simulink model "I2C_MultipleSequence_FinitStateMachine"  (Simulink 6.4)
settings: Solver=FixedStepDiscrete  StartTime=0.0  StopTime=10.0  FixedStep=0.001  RelTol=1e-3
libraries: dsPICdrivers x6, simulink x3
settings Model: Creator=Lubin  LastModifiedBy=Lubin  ProdHWDeviceType=16-bit Generic
settings OptimizationCC: OptimizeModelRefInitCode=on  LifeSpan=1
settings DebuggingCC: MultiTaskDSMMsg=error  MultiTaskCondExecSysMsg=error
settings HardwareCC: ProdBitPerInt=16  ProdWordSize=16  ProdHWDeviceType=16-bit Generic
settings RTWCC: SystemTargetFile=dspic.tlc  TemplateMakefile=dspic_pic30_gcc.tmf  PostCodeGenCommand=dsPIC_Compile()  Description=Embedded Target for Microchip dsPIC (real-time)  ProcessScript=dspic_make_rtw_hook
settings CodeAppCC: IgnoreCustomStorageClasses=off
settings STFCustomTargetCC: TargetFcnLib=ansi_tfl_tmw.mat  GenFloatMathFcnCalls=ANSI_C  ModelReferenceCompliant=off  IncludeMdlTerminateFcn=off  CombineOutputUpdateFcns=on  SuppressErrorStatus=on  IncludeERTFirstTime=on  ERTFirstTimeCompliant=on  ERTCustomFileBanners=on  SupportContinuousTime=off  SupportNonInlinedSFcns=off  SystemTargetFile=dspic.tlc
settings ERTTargetCC: TargetFcnLib=ansi_tfl_tmw.mat  GenFloatMathFcnCalls=ANSI_C  ModelReferenceCompliant=off  IncludeMdlTerminateFcn=off  SuppressErrorStatus=on  IncludeERTFirstTime=on  InlinedParameterPlacement=NonHierarchical  ERTSrcFileBannerTemplate=dsPIC_code_template.cgt  ERTHdrFileBannerTemplate=dsPIC_code_template.cgt  ERTDataSrcFileTemplate=dsPIC_code_template.cgt  ERTDataHdrFileTemplate=dsPIC_code_template.cgt  ERTCustomFileTemplate=dsPIC_main.tlc  InitialValueSource=Model
settings CustomProperty: DataType=string  Value=C:\PROGRA~1\MATLAB\R2007b\bin\win32\gmake

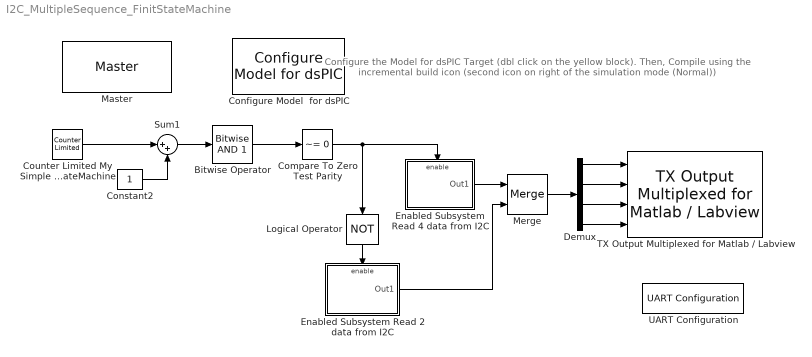
== system I2C_MultipleSequence_FinitStateMachine ==
  note: Configure the Model for dsPIC Target (dbl click on the yellow block).
      | Then, Compile using the incremental build icon
      | (second icon on right of the simulation mode (Normal))
  Bitwise Operator : simulink/Logic and Bit Operations/Bitwise Operator  logicop=AND  UseBitMask=on  BitMask=1  BitMaskRealWorld=Stored Integer
  Compare To Zero Test Parity : simulink/Logic and Bit Operations/Compare To Zero  SystemSampleTime=-1  relop=~=  LogicOutDataTypeMode=uint8  ZeroCross=off
  Configure Model  for dsPIC : dsPICdrivers/Simulink Configuration/Configure Model  for dsPIC
  Constant2 : Constant  Value=1  OutDataTypeMode=uint16  OutDataType=sfix(16)  ConRadixGroup=Use specified scaling  OutScaling=2^0  SampleTime=inf  FramePeriod=inf
  Counter Limited My Simple StateMachine : simulink/Sources/Counter Limited  SystemSampleTime=-1  uplimit=5  tsamp=.001
  Demux : Demux
  Enabled Subsystem Read 2 data from I2C : Subsystem  TreatAsAtomicUnit=on
  Enabled Subsystem Read 4 data from I2C : Subsystem  TreatAsAtomicUnit=on
  Logical Operator : Logic  Orientation=down  Operator=NOT  AllPortsSameDT=off  OutDataTypeMode=Boolean
  Master : dsPICdrivers/Master  Tag=dsPIC_MASTER  Priority=1  TimeStepType=Timer1  picType=30f3012  fcy=2.5e6  Quartz_33f=5e6  PLLActive_33f=off  fcyDesired_33f=0  tmr1="[1  2499  0]"  tmr1Info="Time Step : 0.001  ;   Error : 0%  PR1=2499"  tmr2345="[0  0]"  tmr2345cfg=[-1 -1]  IOautoConf=on  typePort="[ 0   0   0   0   0   0   0   0   0   0   0   0   0   0   0   0   0   0   0   0  20  20   0   0   0   0   0   0   0   0   0   0   0   0   0   0   0   0   0   0   0   0   0   0   0   5   4   0   0   0   0   0   0   0   0   0   0   0   0   0   0   0   0   0   0   0   0   0   0   0   0   0   0   0   0   0   0   0   0   0   0   0   0   0   0   0   0   0   0   0   0   0   0   0   0   0   0   0   0   0   0   0   0   0   0   0   0   0   0   0   0   0 ]"  TRIS="[ 65535  65535  65535  65535  65535  65535  65535 ]"  ADPCFG=0  MasterBusyPort=None  MasterOverloadPort=None  FOSC=HS  TempProtection_33f=TEMP_ON  FPBOR=PBOR_OFF  PWRT=PWRT_OFF  MCLR=MCLR_DIS  PowerSave=off
  Merge : Merge
  Sum1 : Sum  Inputs=|++  OutDataTypeMode=uint16
  TX Output Multiplexed for Matlab / Labview : dsPICdrivers/Serial PORT/TX Output Multiplexed for Matlab // Labview  Tag=dsPIC_TX_Multiplexed  Priority=5  UART=1  CleverSpreadingChk=on  CleverSpreading=1  CHANNEL=[0 1 2 3]  BUFFERSIZE=16  CHANNELBLOCKED=[]  CHANNELBLOCKED_BITEWISE=0  Status=OK
  UART Configuration : dsPICdrivers/Serial PORT/UART Configuration  Tag=dsPIC_config_UART  Priority=2  UART=1  proposed_BAUD=38400  ALT_TX_RX=on  TXInterruptPri=1  InterruptTxWhen=on TxBUF becoming empty  TXEN=on  RXInterruptPri=1  BAUD=38400  UxBRG=3  Info="UxBRG = 3   ||  Real Baud : 39063   ||  % error : 1.7253  ||  max 3.9063 Bytes / Step"  RealBaud=0
  wires:
  Counter Limited My Simple StateMachine/1 -> Sum1/1
  Constant2/1 -> Sum1/2
  Sum1/1 -> Bitwise Operator/1
  Bitwise Operator/1 -> Compare To Zero Test Parity/1
  Compare To Zero Test Parity/1 -> Enabled Subsystem Read 4 data from I2C/Enable, Logical Operator/1
  Logical Operator/1 -> Enabled Subsystem Read 2 data from I2C/Enable
  Enabled Subsystem Read 4 data from I2C/1(Out1) -> Merge/1
  Enabled Subsystem Read 2 data from I2C/1(Out1) -> Merge/2
  Merge/1 -> Demux/1
  Demux/1 -> TX Output Multiplexed for Matlab / Labview/1
  Demux/2 -> TX Output Multiplexed for Matlab / Labview/2
  Demux/3 -> TX Output Multiplexed for Matlab / Labview/3
  Demux/4 -> TX Output Multiplexed for Matlab / Labview/4

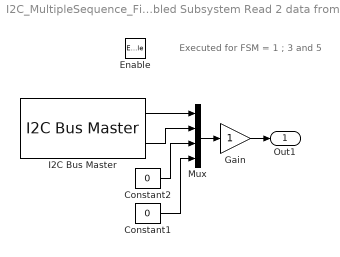
== system I2C_MultipleSequence_FinitStateMachine/Enabled Subsystem Read 2 data from I2C ==
  note: Executed for FSM = 1 ; 3 and 5
  Enable : EnablePort
  Constant1 : Constant  Value=0  OutDataType=sfix(16)  ConRadixGroup=Use specified scaling  OutScaling=2^0  SampleTime=inf  FramePeriod=inf
  Constant2 : Constant  Value=0  OutDataType=sfix(16)  ConRadixGroup=Use specified scaling  OutScaling=2^0  SampleTime=inf  FramePeriod=inf
  Gain : Gain
  I2C Bus Master : dsPICdrivers/BUS I2C/I2C Bus Master  Tag=dsPIC_I2C_Master  NumI2C=1  Sequence='S A100 R R P'  InitializeOnceOnly=When PIC is initialized (only once)  Enable=off  WaitAfterEnable=1  Disable=off  AdressNbrBits=7 bits  I2CBusFreq=227  SlewRate=off  SMBUSThreshold=off  OutputErrorFlag=off  SampleTime=-1  OrderingInOutPopup=None  Info=Fscl = 10.8578 KHz
  Mux : Mux
  Out1 : Outport
  wires:
  Mux/1 -> Gain/1
  I2C Bus Master/1 -> Mux/1
  I2C Bus Master/2 -> Mux/2
  Constant2/1 -> Mux/3
  Constant1/1 -> Mux/4
  Gain/1 -> Out1/1

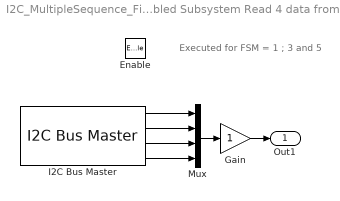
== system I2C_MultipleSequence_FinitStateMachine/Enabled Subsystem Read 4 data from I2C ==
  note: Executed for FSM = 1 ; 3 and 5
  Enable : EnablePort
  Gain : Gain
  I2C Bus Master : dsPICdrivers/BUS I2C/I2C Bus Master  Tag=dsPIC_I2C_Master  NumI2C=1  Sequence='S A100 R R R R P'  InitializeOnceOnly=When PIC is initialized (only once)  Enable=off  WaitAfterEnable=1  Disable=off  AdressNbrBits=7 bits  I2CBusFreq=227  SlewRate=off  SMBUSThreshold=off  OutputErrorFlag=off  SampleTime=-1  OrderingInOutPopup=None  Info=Fscl = 10.8578 KHz
  Mux : Mux
  Out1 : Outport
  wires:
  I2C Bus Master/1 -> Mux/1
  I2C Bus Master/2 -> Mux/2
  I2C Bus Master/3 -> Mux/3
  I2C Bus Master/4 -> Mux/4
  Mux/1 -> Gain/1
  Gain/1 -> Out1/1
